simulink model "UAV_SIMULATOR_CA_2021a"  (R2024a)
settings: Solver=FixedStepAuto  StartTime=0.0  StopTime=tf_echelons  FixedStep=0.002  RelTol=1e-4
values from neighbouring files (symbols this model uses):
  Beta_OPT = [Beta, Z_max: 0.1*pi/180: betaf]    [UAV_SIMULATOR_MAIN_0.m]
  betaf = 20*pi/180 +betai    (= 0.660268528005)    [UAV_SIMULATOR_MAIN_0.m]
  betai = 17.8306*pi/180    (= 0.311202677606)    [UAV_SIMULATOR_MAIN_0.m]
  Bp_offset = 0.06    [UAV_SIMULATOR_MAIN_0.m]
  CDy = data(1)    [Aero_initial.m]    (also in FunLagragian.m; UAV_SIMULATOR_MAIN_0.m = 1; costFunction.m; nonLinearConstraints.m)
  CLOSED_LOOP_ESCs = 1    [UAV_SIMULATOR_MAIN_0.m]
  cQ = 2.1113*1e-08    (= 2.1113e-08)    [UAV_SIMULATOR_MAIN_0.m]
  cQ_Magnus = 0.5*S/2*RM^3*Cf    (= 4.804078125e-10)    [UAV_SIMULATOR_MAIN_0.m]
  cT = 2.4815e-6    (= 2.4815e-06)    [UAV_SIMULATOR_MAIN_0.m]
  cT_1_6 = 2.1030e-06    (= 2.103e-06)    [UAV_SIMULATOR_MAIN_0.m]
  D_PQR_PX4 = diag([D_ROLL D_PITCH D_YAW])    [UAV_SIMULATOR_MAIN_0.m]
  ethaf = 25*pi/180    (= 0.436332312999)    [UAV_SIMULATOR_MAIN_0.m]
  ethai = 0 *pi/180    (= 0)    [UAV_SIMULATOR_MAIN_0.m]
  F_fric = 0.5    [UAV_SIMULATOR_MAIN_0.m]
  Fa_L_int = Rmat*(FaG_int+FaG_int_d)    [UAV_SIMULATOR_MAIN_0.m]
  g = data(7)    [FunLagragian.m]    (also in UAV_SIMULATOR_MAIN_0.m = 9.81; costFunction.m; nonLinearConstraints.m; runOptimizationHelper.m = comp(7))
  I_PQR_PX4 = diag([I_ROLL I_PITCH I_YAW])    [UAV_SIMULATOR_MAIN_0.m]
  initial_attitude_condition = 1*[0 0 pi]    [UAV_SIMULATOR_MAIN_0.m]
  initial_pos_conditions = [ri*cos(betai) 0 ri*sin(betai) + Bp_offset]    [UAV_SIMULATOR_MAIN_0.m]
  Jr = 1.2991*1e-05    (= 1.2991e-05)    [UAV_SIMULATOR_MAIN_0.m]
  Jr_Magnus = JM1(2,2)    [UAV_SIMULATOR_MAIN_0.m]
  K_DI_int = [diag([k_r(1), k_etha(1), k_beta(1)]), diag([k_r(2), k_etha(2), k_beta(2)]), diag([k_r(3), k_etha(3), k_beta(3)])]    [UAV_SIMULATOR_MAIN_0.m]
  K_PQR_PX4 = 1*diag([0.8 1.35 1])    [UAV_SIMULATOR_MAIN_0.m]
  km = 1/Kv_motor_rad    (= 0.00545674090601)    [UAV_SIMULATOR_MAIN_0.m]
  L = lqr(A,B,Q_beta,R_beta)    [UAV_SIMULATOR_MAIN_0.m]
  L_mot = 1.0000e-04    (= 0.0001)    [UAV_SIMULATOR_MAIN_0.m]
  LM = 0.28*2    (= 0.56)    [UAV_SIMULATOR_MAIN_0.m]
  m = data(6)    [FunLagragian.m]    (also in UAV_SIMULATOR_MAIN_0.m = 1.746; costFunction.m; nonLinearConstraints.m; runOptimizationHelper.m = comp(6))
  m_M1 = 0.049    [UAV_SIMULATOR_MAIN_0.m]
  m_M2 = 0.049    [UAV_SIMULATOR_MAIN_0.m]
  m_w = 0.0481    [UAV_SIMULATOR_MAIN_0.m]    (also in nonLinearConstraints.m = data(9); runOptimizationHelper.m = comp(9))
  max_angle = max_angle_deg*pi/180    (= 0.610865238198)    [UAV_SIMULATOR_MAIN_0.m]
  nb_battery_cells = 4    [UAV_SIMULATOR_MAIN_0.m]
  P_ATTITUDE_PX4 = diag([10 10 2.8])    [UAV_SIMULATOR_MAIN_0.m]
  P_PQR_PX4 = diag([P_ROLL P_PITCH P_YAW])    [UAV_SIMULATOR_MAIN_0.m]
  PX4_attitude_loop_frequency = 250    [UAV_SIMULATOR_MAIN_0.m]
  PX4_rate_loop_frequency = 500    [UAV_SIMULATOR_MAIN_0.m]
  R = data(4)    [Aero_initial.m]    (also in UAV_SIMULATOR_MAIN_0.m = 0.07)
  R_bat = 0.024    [UAV_SIMULATOR_MAIN_0.m]
  rf = 1.5    [UAV_SIMULATOR_MAIN_0.m]
  rho_air = data(8)    [FunLagragian.m]    (also in UAV_SIMULATOR_MAIN_0.m = 1.293; costFunction.m; nonLinearConstraints.m; runOptimizationHelper.m = comp(8))
  ri = 0.490142    [UAV_SIMULATOR_MAIN_0.m]
  RM = data(4)    [FunLagragian.m]    (also in UAV_SIMULATOR_MAIN_0.m = 0.0275; costFunction.m; nonLinearConstraints.m; runOptimizationHelper.m = comp(4))
  S = data(3)    [Aero_initial.m]    (also in FunLagragian.m; UAV_SIMULATOR_MAIN_0.m = 0.0308; costFunction.m; nonLinearConstraints.m)
  s_M1D = [0, LM/4, 0]'    [UAV_SIMULATOR_MAIN_0.m]
  s_M2D = [0, -LM/4, 0]'    [UAV_SIMULATOR_MAIN_0.m]
  Slat = data(2)    [Aero_initial.m]    (also in FunLagragian.m; UAV_SIMULATOR_MAIN_0.m = 0.00237582944428; costFunction.m; nonLinearConstraints.m)
  state_int = [0 0 0 initial_attitude_condition 0 0 0 initial_attitude_quaternion_condition]    [UAV_SIMULATOR_MAIN_0.m]
  T0 = 1.5    [UAV_SIMULATOR_MAIN_0.m]
  t0 = 0    [UAV_SIMULATOR_MAIN_0.m]
  t1 = t0 + 15    (= 15)    [UAV_SIMULATOR_MAIN_0.m]
  t1T = t1/10    (= 1.5)    [UAV_SIMULATOR_MAIN_0.m]
  t2 = t1 + 15    (= 30)    [UAV_SIMULATOR_MAIN_0.m]    (also in plot_test.m = Simulation_Data.time)
  t2T = t2 + 9*t1/10    (= 43.5)    [UAV_SIMULATOR_MAIN_0.m]
  t3 = t2 + 15    (= 45)    [UAV_SIMULATOR_MAIN_0.m]
  tau_ur_model = 0.001    [UAV_SIMULATOR_MAIN_0.m]
  Tf = 1.5    [UAV_SIMULATOR_MAIN_0.m]
  Ti = 0    [UAV_SIMULATOR_MAIN_0.m]
  Ts = 0.02    [UAV_SIMULATOR_MAIN_0.m]
  U_sat = 3.7*nb_battery_cells    (= 14.8)    [UAV_SIMULATOR_MAIN_0.m]
  ViconTracker_noise_mean = 0.00001    (= 1e-05)    [UAV_SIMULATOR_MAIN_0.m]
  ViconTracker_noise_variance = 0.000001    (= 1e-06)    [UAV_SIMULATOR_MAIN_0.m]
  vitesse_vent = [0, 0, 0]'    [UAV_SIMULATOR_MAIN_0.m]
  vmag = 0    [UAV_SIMULATOR_MAIN_0.m]
  vx_wind = [vwind(1,1:t_winddirc_change/dt-1) vx_inter vwind(1,(t_winddirc_change+1)/dt +1:final_time/dt+1)*cos(10*pi/180)]    [UAV_SIMULATOR_MAIN_0.m]
  vy_wind = [zeros(1,t_winddirc_change/dt-1) vy_inter vwind(1,(t_winddirc_change+1)/dt +1:final_time/dt+1)*sin(10*pi/180)]    [UAV_SIMULATOR_MAIN_0.m]
  wind_turb = 1    [UAV_SIMULATOR_MAIN_0.m]
  wn_beta = 2    [UAV_SIMULATOR_MAIN_0.m]
  wn_etha = 2    [UAV_SIMULATOR_MAIN_0.m]
  wn_r = 2    [UAV_SIMULATOR_MAIN_0.m]
  X0 = 4    [UAV_SIMULATOR_MAIN_0.m]    (also in runOptimizationHelper.m = data(19))
  X1 = min(X1,8)    [Aero_initial.m]    (also in UAV_SIMULATOR_MAIN_0.m = [X1, X1(end)])
undefined symbols (not defined in the file or in its folder): DiscIntNeverNeededParam, PWM_data_map
libraries: simulink x23, slpidlib x5, eeGeneralControl x3, simulink_extras x1
(part 2 of 3)

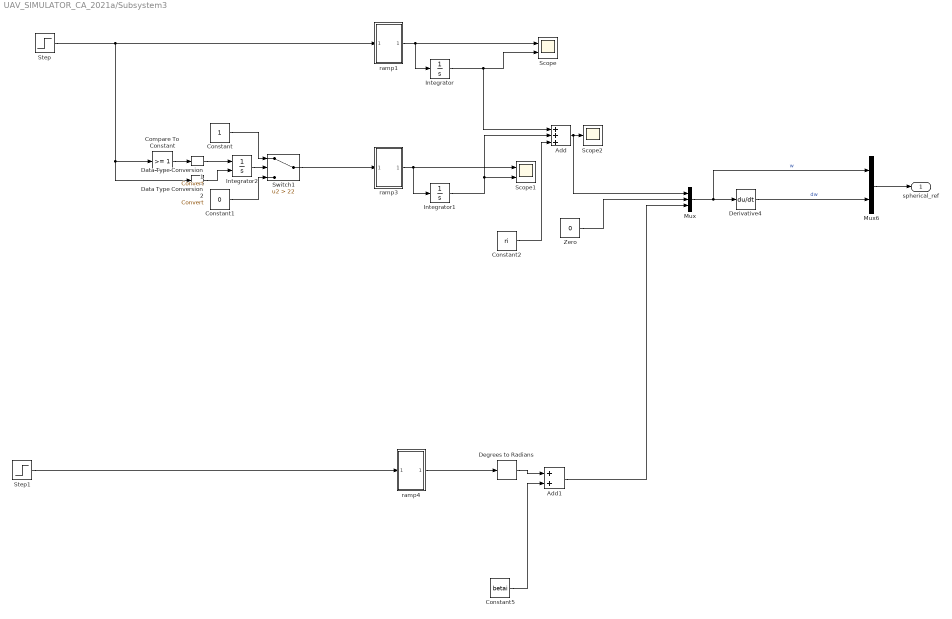
== system UAV_SIMULATOR_CA_2021a/Subsystem3 ==
  Add : Sum  Inputs=+++
  Add1 : Sum
  Compare To Constant : simulink/Logic and Bit Operations/Compare To Constant  relop=>=  const=1  OutDataTypeStr=uint8
  Constant : Constant
  Constant1 : Constant  Value=0
  Constant2 : Constant  Value=ri
  Constant5 : Constant  Value=betai
  Data Type Conversion1 : DataTypeConversion  SaturateOnIntegerOverflow=off  RndMeth=Floor
  Data Type Conversion2 : DataTypeConversion  SaturateOnIntegerOverflow=off  RndMeth=Floor
  Degrees to Radians : simulink_extras/Transformations/Degrees to Radians
  Derivative4 : Derivative
  Integrator : Integrator
  Integrator1 : Integrator
  Integrator2 : Integrator  ExternalReset=falling
  Mux : Mux  Inputs=3
  Mux6 : Mux  Inputs=2
  Scope : Scope  NumInputPorts=2
  Scope1 : Scope  NumInputPorts=2
  Scope2 : Scope
  Step : Step  Time=0  SampleTime=0
  Step1 : Step  Time=0  SampleTime=0
  Switch1 : Switch  Criteria=u2 > Threshold  Threshold=22  SaturateOnIntegerOverflow=off  InputSameDT=off
  Zero : Constant  Value=0  OutDataTypeStr=Inherit: Inherit via back propagation
  ramp1 : Subsystem  mask{tf1=4, tf2=8, tf3=4, g1=(1/12)/4, g2=(1/12)/4}
      mask prompts: tf1 "temps fin rampe montante"; tf2 "temps fin constante"; tf3 "temps fin rampe descendente"; g1 "gain rampe 1"; g2 "gain rampe 2"
  ramp3 : Subsystem  mask{tf1=4, tf2=8, tf3=4, g1=-(1/12)/4, g2=-(1/12)/4}
      mask prompts: tf1 "temps fin rampe montante"; tf2 "temps fin constante"; tf3 "temps fin rampe descendente"; g1 "gain rampe 1"; g2 "gain rampe 2"
  ramp4 : Subsystem  mask{tf1=10, tf2=26, tf3=10, g1=15/10, g2=15/10}
      mask prompts: tf1 "temps fin rampe montante"; tf2 "temps fin constante"; tf3 "temps fin rampe descendente"; g1 "gain rampe 1"; g2 "gain rampe 2"
  spherical_ref : Outport
  wires:
  Degrees to Radians/1 -> Add1/1
  ramp3/1(Out1) -> Scope1/1, Integrator1/1
  ramp4/1(Out1) -> Degrees to Radians/1
  Constant1/1 -> Switch1/3
  Constant/1 -> Switch1/1
  ramp1/1(Out1) -> Scope/1, Integrator/1
  Add/1 -> Mux/1, Scope2/1
  Compare To Constant/1 -> Data Type Conversion1/1
  Switch1/1 -> ramp3/1(In1)
  Integrator2/1 -> Switch1/2
  Data Type Conversion2/1 -> Integrator2/2
  Data Type Conversion1/1 -> Integrator2/1
  Integrator1/1 -> Scope1/2, Add/2
  Step/1 -> ramp1/1(In1), Compare To Constant/1, Data Type Conversion2/1
  Constant2/1 -> Add/3
  Integrator/1 -> Scope/2, Add/1
  Constant5/1 -> Add1/2
  Add1/1 -> Mux/3
  Zero/1 -> Mux/2
  Mux6/1 -> spherical_ref/1
  Mux/1 -> Derivative4/1, Mux6/1  "w"
  Derivative4/1 -> Mux6/2  "dw"
  Step1/1 -> ramp4/1(In1)

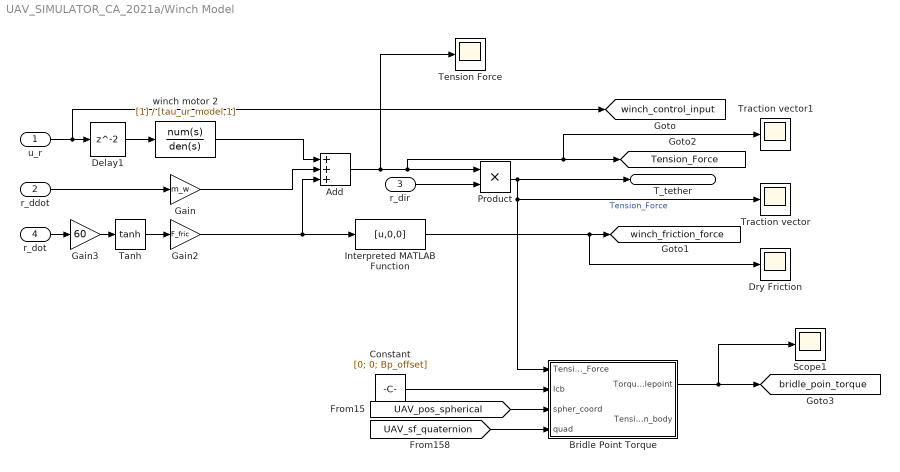
== system UAV_SIMULATOR_CA_2021a/Winch Model ==
  u_r : Inport
  r_ddot : Inport  Port=2
  r_dir : Inport  Port=3
  r_dot : Inport  Port=4
  Add : Sum  Inputs=+++
  Bridle Point Torque : MATLAB Function  TreatAsAtomicUnit=on
  Constant : Constant  Value=[0; 0; Bp_offset]
  Delay1 : Delay  SampleTime=Ts
  Dry Friction : Scope
  Gain : Gain  Gain=m_w
  Gain2 : Gain  Gain=F_fric
  Gain3 : Gain  Gain=60
  Interpreted MATLAB Function : MATLABFcn  MATLABFcn=[u,0,0]
  Product : Product
  Scope1 : Scope
  Tanh : Trigonometry  Operator=tanh
  Tension Force : Scope
  Traction vector : Scope
  Traction vector1 : Scope
  winch motor 2 : TransferFcn  Denominator=[tau_ur_model,1]
  T_tether : Outport
  tag scope: Tension_Force=global, bridle_poin_torque=global, winch_control_input=global, winch_friction_force=global
  wires:
  Gain/1 -> Add/2
  Product/1 -> T_tether/1, Traction vector/1, Bridle Point Torque/1(Tension_Force)  "Tension_Force"
  Add/1 -> Tension Force/1, Traction vector1/1, [Tension_Force], Product/1
  r_dir/1 -> Product/2
  r_dot/1 -> Gain3/1
  Interpreted MATLAB Function/1 -> Dry Friction/1, [winch_friction_force]
  Tanh/1 -> Gain2/1
  Gain3/1 -> Tanh/1
  r_ddot/1 -> Gain/1
  u_r/1 -> [winch_control_input], Delay1/1
  Gain2/1 -> Interpreted MATLAB Function/1, Add/3
  Delay1/1 -> winch motor 2/1
  winch motor 2/1 -> Add/1
  Constant/1 -> Bridle Point Torque/2(lcb)
  [UAV_pos_spherical] -> Bridle Point Torque/3(spher_coord)
  [UAV_sf_quaternion] -> Bridle Point Torque/4(quad)
  Bridle Point Torque/1(Torque_bridlepoint) -> Scope1/1, [bridle_poin_torque]

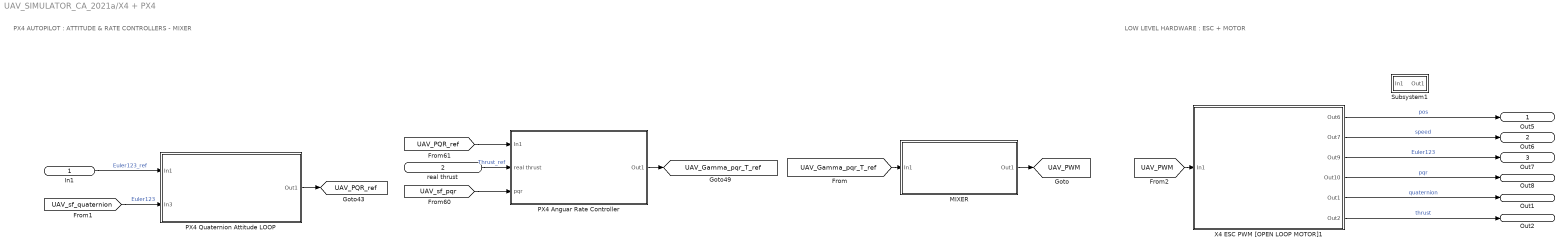
== system UAV_SIMULATOR_CA_2021a/X4 + PX4  ==
  note: LOW LEVEL HARDWARE : ESC + MOTOR
  note: PX4 AUTOPILOT : ATTITUDE & RATE CONTROLLERS - MIXER
  In1 : Inport
  real thrust : Inport  Port=2
  MIXER : Subsystem
  PX4 Anguar Rate Controller : Subsystem
  PX4 Quaternion Attitude LOOP : Subsystem
  Subsystem1 : Subsystem
  X4 ESC PWM [OPEN LOOP MOTOR]1 : Subsystem
  Out5 : Outport
  Out6 : Outport  Port=2
  Out7 : Outport  Port=3
  Out8 : Outport  Port=4
  Out1 : Outport  Port=5
  Out2 : Outport  Port=6
  tag scope: UAV_Gamma_pqr_T_ref=global, UAV_PQR_ref=global, UAV_PWM=global
  wires:
  [UAV_sf_quaternion] -> PX4 Quaternion Attitude LOOP/2(In3)  "Euler123"
  PX4 Quaternion Attitude LOOP/1(Out1) -> [UAV_PQR_ref]
  [UAV_Gamma_pqr_T_ref] -> MIXER/1(In1)
  [UAV_sf_pqr] -> PX4 Anguar Rate Controller/3(pqr)
  MIXER/1(Out1) -> [UAV_PWM]
  real thrust/1 -> PX4 Anguar Rate Controller/2(real thrust)  "Thrust_ref"
  In1/1 -> PX4 Quaternion Attitude LOOP/1(In1)  "Euler123_ref"
  [UAV_PQR_ref] -> PX4 Anguar Rate Controller/1(In1)
  PX4 Anguar Rate Controller/1(Out1) -> [UAV_Gamma_pqr_T_ref]
  X4 ESC PWM [OPEN LOOP MOTOR]1/3(Out9) -> Out7/1  "Euler123"
  X4 ESC PWM [OPEN LOOP MOTOR]1/2(Out7) -> Out6/1  "speed"
  [UAV_PWM] -> X4 ESC PWM [OPEN LOOP MOTOR]1/1(In1)
  X4 ESC PWM [OPEN LOOP MOTOR]1/4(Out10) -> Out8/1  "pqr"
  X4 ESC PWM [OPEN LOOP MOTOR]1/5(Out1) -> Out1/1  "quaternion"
  X4 ESC PWM [OPEN LOOP MOTOR]1/6(Out2) -> Out2/1  "thrust"
  X4 ESC PWM [OPEN LOOP MOTOR]1/1(Out6) -> Out5/1  "pos"

== system UAV_SIMULATOR_CA_2021a/r_ref ==
  Add : Sum  Inputs=+++
  Add1 : Sum  Inputs=+++
  Add3 : Sum
  Add4 : Sum  Inputs=+++
  Ramp : simulink/Sources/Ramp  slope=(Tf-Ti)/(t1T-t0)  start=t0  InitialOutput=Ti
  Ramp2 : simulink/Sources/Ramp  slope=-(Tf-Ti)/(t1T-t0)  start=t1T  InitialOutput=-Tf
  Ramp3 : simulink/Sources/Ramp  slope=(Ti-Tf)/(t3-t2T)  start=t2T  InitialOutput=Tf
  Ramp5 : simulink/Sources/Ramp  slope=-(Ti-Tf)/(t3-t2T)  start=t3  InitialOutput=-Ti  VectorParams1D=off
  Step : Step  Time=t2T  Before=Tf  After=0  SampleTime=0
  Step2 : Step  Time=t1T  Before=-Tf  After=0  SampleTime=0
  Step4 : Step  Time=t1T  Before=Tf  After=0  SampleTime=0
  Step6 : Step  Time=t2T  Before=Ti-Tf  After=Ti  SampleTime=0
  T_ref : Outport
  wires:
  Add3/1 -> Add4/2
  Ramp/1 -> Add/1
  Step6/1 -> Add1/3
  Ramp2/1 -> Add/2
  Ramp3/1 -> Add1/1
  Add1/1 -> Add4/3
  Add4/1 -> T_ref/1
  Step/1 -> Add3/1
  Ramp5/1 -> Add1/2
  Step2/1 -> Add3/2
  Step4/1 -> Add/3
  Add/1 -> Add4/1

== system UAV_SIMULATOR_CA_2021a/ramp4 ==
  In1 : Inport
  Add : Sum
  Compare To Constant : simulink/Logic and Bit Operations/Compare To Constant  relop=>=  const=1  OutDataTypeStr=uint8
  Constant : Constant  Value=-1
  Constant1 : Constant  Value=0
  Data Type Conversion1 : DataTypeConversion  SaturateOnIntegerOverflow=off  RndMeth=Floor
  Data Type Conversion2 : DataTypeConversion  SaturateOnIntegerOverflow=off  RndMeth=Floor
  Gain : Gain  Gain=g1
  Gain2 : Gain  Gain=g2
  Integrator : Integrator  ExternalReset=falling
  Integrator1 : Integrator  ExternalReset=falling
  Switch : Switch  Criteria=u2 > Threshold  Threshold=tf2+tf1  SaturateOnIntegerOverflow=off  InputSameDT=off
  Switch1 : Switch  Criteria=u2 > Threshold  Threshold=tf1  SaturateOnIntegerOverflow=off  InputSameDT=off
  Switch2 : Switch  Criteria=u2 > Threshold  Threshold=tf3+tf2+tf1  SaturateOnIntegerOverflow=off  InputSameDT=off
  Out1 : Outport
  wires:
  Compare To Constant/1 -> Data Type Conversion1/1
  Integrator/1 -> Switch1/2, Switch2/2, Switch/2
  In1/1 -> Data Type Conversion2/1, Compare To Constant/1
  Data Type Conversion1/1 -> Integrator/1, Switch1/3
  Data Type Conversion2/1 -> Integrator1/2, Integrator/2
  Constant/1 -> Switch/1
  Switch2/1 -> Gain2/1
  Constant1/1 -> Switch/3, Switch2/1, Switch1/1
  Switch1/1 -> Gain/1
  Integrator1/1 -> Out1/1
  Gain2/1 -> Add/2
  Gain/1 -> Add/1
  Add/1 -> Integrator1/1
  Switch/1 -> Switch2/3

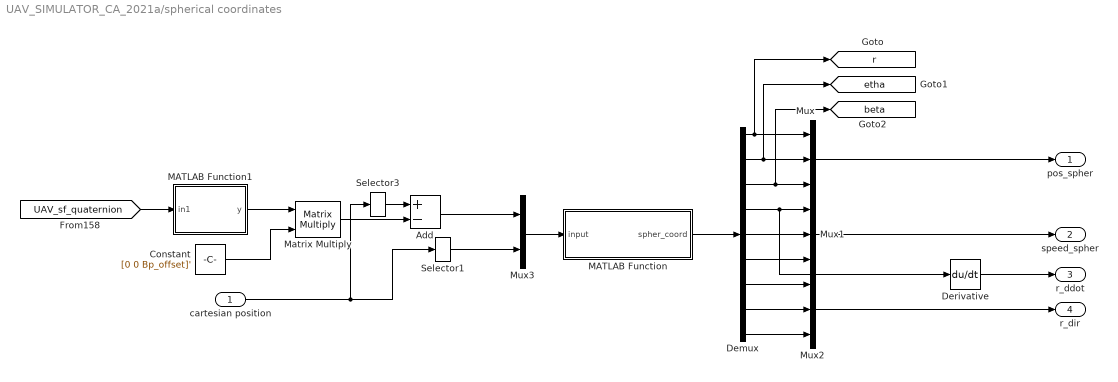
== system UAV_SIMULATOR_CA_2021a/spherical coordinates ==
  "cartesian position " : Inport
  Add : Sum  Inputs=+-
  Constant : Constant  Value=[0 0 Bp_offset]'
  Demux : Demux  Outputs=9
  Derivative : Derivative
  MATLAB Function : MATLAB Function  TreatAsAtomicUnit=on
  MATLAB Function1 : MATLAB Function  TreatAsAtomicUnit=on
  Matrix Multiply : Product  Multiplication=Matrix(*)
  Mux : Mux  Inputs=3
  Mux1 : Mux  Inputs=3
  Mux2 : Mux  Inputs=3
  Mux3 : Mux  Inputs=2
  Selector1 : Selector  InputPortWidth=6  IndexOptions=Index vector (dialog)  Indices=[4:6]  OutputSizes=1
  Selector3 : Selector  InputPortWidth=6  IndexOptions=Index vector (dialog)  Indices=[1:3]  OutputSizes=1
  pos_spher : Outport
  speed_spher : Outport  Port=2
  r_ddot : Outport  Port=3
  r_dir : Outport  Port=4
  tag scope: beta=global, etha=global, r=global
  wires:
  MATLAB Function/1(spher_coord) -> Demux/1
  Demux/1 -> [r], Mux/1
  Demux/2 -> [etha], Mux/2
  Demux/3 -> [beta], Mux/3
  Demux/5 -> Mux1/2
  Demux/6 -> Mux1/3
  Demux/4 -> Derivative/1, Mux1/1
  Mux/1 -> pos_spher/1
  Mux1/1 -> speed_spher/1
  Derivative/1 -> r_ddot/1
  Demux/7 -> Mux2/1
  Demux/8 -> Mux2/2
  Demux/9 -> Mux2/3
  Mux2/1 -> r_dir/1
  Selector3/1 -> Add/1
  "cartesian position "/1 -> Selector1/1, Selector3/1
  Constant/1 -> Matrix Multiply/2
  Matrix Multiply/1 -> Add/2
  MATLAB Function1/1(y) -> Matrix Multiply/1
  [UAV_sf_quaternion] -> MATLAB Function1/1(in1)
  Selector1/1 -> Mux3/2
  Add/1 -> Mux3/1
  Mux3/1 -> MATLAB Function/1(input)

== system UAV_SIMULATOR_CA_2021a/Aerodynamic Forces/Magnus_Actuator ==
  In1 : Inport
  PID Controller1 : slpidlib/PID Controller  Controller=PID  Form=Parallel  TimeDomain=Continuous-time  UseExternalTs=off  SampleTime=-1  IntegratorMethod=Forward Euler  FilterMethod=Forward Euler  ControllerParametersSource=internal  P=0.01  I=0.4  UseKiTs=off  D=0  UseExternalDerivativeSource=off  N=100  UseFilter=on  TunerSelectOption=Transfer Function Based (PID Tuner App)  InitialConditionSource=internal  InitialConditionForIntegrator=0  InitialConditionForFilter=0  DifferentiatorICPrevScaledInput=0  ExternalReset=none  TrackingMode=off  Kt=1  LimitOutput=off  SatLimitsSource=internal  UpperSaturationLimit=inf  LowerSaturationLimit=-inf  LinearizeAsGain=on  AntiWindupMode=none  Kb=1  LimitIntegrator=off  UpperIntegratorSaturationLimit=inf  LowerIntegratorSaturationLimit=-inf  POutMin=[]  POutMax=[]  IOutMin=[]  IOutMax=[]  DOutMin=[]  DOutMax=[]  NOutMin=[]  NOutMax=[]  SumOutMin=[]  SumOutMax=[]  SaturationOutMin=[]  SaturationOutMax=[]  PParamMin=[]  PParamMax=[]  IParamMin=[]  IParamMax=[]  DParamMin=[]  DParamMax=[]  NParamMin=[]  NParamMax=[]  KbParamMin=[]  KbParamMax=[]  KtParamMin=[]  KtParamMax=[]  KbOutMin=[]  KbOutMax=[]  KtOutMin=[]  KtOutMax=[]  IntegratorOutMin=[]  IntegratorOutMax=[]  FilterOutMin=[]  FilterOutMax=[]  SumI1OutMin=[]  SumI1OutMax=[]  SumI2OutMin=[]  SumI2OutMax=[]  SumI3OutMin=[]  SumI3OutMax=[]  SumI4OutMin=[]  SumI4OutMax=[]  SumDOutMin=[]  SumDOutMax=[]  DifferentiatorOutMin=[]  DifferentiatorOutMax=[]  FilterDiffOutCoefMin=[]  FilterDiffOutCoefMax=[]  ReciprocalOutMin=[]  ReciprocalOutMax=[]  SumDenOutMin=[]  SumDenOutMax=[]  SumNumOutMin=[]  SumNumOutMax=[]  DivideOutMin=[]  DivideOutMax=[]  UdiffTsProdOutMin=[]  UdiffTsProdOutMax=[]  NTsProdOutMin=[]  NTsProdOutMax=[]  UintegralTsProdOutMin=[]  UintegralTsProdOutMax=[]  UngainTsProdOutMin=[]  UngainTsProdOutMax=[]  ClampingZeroOutDataTypeStr=Inherit: Inherit via back propagation  ClampingZeroOutMin=[]  ClampingZeroOutMax=[]  FilterDenConstantOutDataTypeStr=Inherit: Inherit via back propagation  FilterDenConstantOutMin=[]  FilterDenConstantOutMax=[]  PCopyOutDataTypeStr=Inherit: Inherit via back propagation  PCopyOutMin=[]  PCopyOutMax=[]  NCopyOutDataTypeStr=Inherit: Inherit via back propagation  NCopyOutMin=[]  NCopyOutMax=[]  IntegratorContinuousStateAttributes=''  IntegratorStateMustResolveToSignalObject=off  IntegratorRTWStateStorageClass=Auto  FilterContinuousStateAttributes=''  FilterStateMustResolveToSignalObject=off  FilterRTWStateStorageClass=Auto  ParallelPVariant=InternalParameters  IdealPVariant=Disabled  IVariant=InternalParameters  DVariant=InternalParameters  IntegratorVariant=Continuous  SatVariant=Disabled  AWVariant=Passthrough  PCopyVariant=Disabled  TRVariant=Disabled  FdbkBlocksVariant=Forward  IdealPFdbkVariant=Disabled  SatFdbkVariant=Disabled  DerivativeFilterVariant=ContFilter  NVariant=InternalParameters  NCopyVariant=Disabled  FilterICVariant=InternalICsFilter  IntegratorICVariant=InternalICs  ExternalResetVariant=Disabled  TRSumVariant=Passthrough  SumFdbkVariant=Disabled  SumVariant=Sum_PID  TsampFilterVariant=InternalTs  TsampNgainVariant=Passthrough  TsampIntegralVariant=Disabled_SignalSpec  ExternalSaturationOutDataTypeStr=Inherit: Same as second input  DerivativeSourceVariant=ErrorSignal
  Scope : Scope
  Subsystem : Subsystem
  Sum7 : Sum  Inputs=|+-
  motor_speed : Outport
  wires:
  Sum7/1 -> PID Controller1/1
  In1/1 -> Scope/1, Sum7/1  "rotation_speed"
  PID Controller1/1 -> Subsystem/1(In1)
  Subsystem/1(Out1) -> motor_speed/1, Sum7/2  "motor_speed"

== system UAV_SIMULATOR_CA_2021a/Subsystem1/beta_ref ==
  Add10 : Sum
  Add11 : Sum  Inputs=+++
  Add8 : Sum  Inputs=+++
  Add9 : Sum  Inputs=+++
  Ramp10 : simulink/Sources/Ramp  slope=(betai-betaf)/(t3-t2)  start=t2  InitialOutput=betaf
  Ramp11 : simulink/Sources/Ramp  slope=-(betai-betaf)/(t3-t2)  start=t3  InitialOutput=-betai  VectorParams1D=off
  Ramp8 : simulink/Sources/Ramp  slope=(betaf-betai)/(t1-t0)  start=t0  InitialOutput=betai
  Ramp9 : simulink/Sources/Ramp  slope=-(betaf-betai)/(t1-t0)  start=t1  InitialOutput=-betaf
  Step10 : Step  Time=t1  Before=betaf  After=0  SampleTime=0
  Step11 : Step  Time=t2  Before=betai-betaf  After=betai  SampleTime=0
  Step8 : Step  Time=t2  Before=betaf  After=0  SampleTime=0
  Step9 : Step  Time=t1  Before=-betaf  After=0  SampleTime=0
  beta-ref : Outport
  wires:
  Ramp10/1 -> Add9/1
  Ramp11/1 -> Add9/2
  Ramp8/1 -> Add8/1
  Step11/1 -> Add9/3
  Add9/1 -> Add11/3
  Add11/1 -> beta-ref/1
  Step10/1 -> Add8/3
  Step8/1 -> Add10/1
  Add10/1 -> Add11/2
  Step9/1 -> Add10/2
  Add8/1 -> Add11/1
  Ramp9/1 -> Add8/2

== system UAV_SIMULATOR_CA_2021a/Subsystem1/etha_ref1 ==
  Add10 : Sum
  Add11 : Sum  Inputs=+++
  Add8 : Sum  Inputs=+++
  Add9 : Sum  Inputs=+++
  Ramp10 : simulink/Sources/Ramp  slope=(ethai-ethaf)/(t3-t2)  start=t2  InitialOutput=ethaf
  Ramp11 : simulink/Sources/Ramp  slope=-(ethai-ethaf)/(t3-t2)  start=t3  InitialOutput=-ethai  VectorParams1D=off
  Ramp8 : simulink/Sources/Ramp  slope=(ethaf-ethai)/(t1-t0)  start=t0  InitialOutput=ethai
  Ramp9 : simulink/Sources/Ramp  slope=-(ethaf-ethai)/(t1-t0)  start=t1  InitialOutput=-ethaf
  Step10 : Step  Time=t1  Before=ethaf  After=0  SampleTime=0
  Step11 : Step  Time=t2  Before=ethai-ethaf  After=ethai  SampleTime=0
  Step8 : Step  Time=t2  Before=ethaf  After=0  SampleTime=0
  Step9 : Step  Time=t1  Before=-ethaf  After=0  SampleTime=0
  beta-ref : Outport
  wires:
  Ramp10/1 -> Add9/1
  Ramp11/1 -> Add9/2
  Ramp8/1 -> Add8/1
  Step11/1 -> Add9/3
  Add9/1 -> Add11/3
  Add11/1 -> beta-ref/1  "etha_ref"
  Step10/1 -> Add8/3
  Step8/1 -> Add10/1
  Add10/1 -> Add11/2
  Step9/1 -> Add10/2
  Add8/1 -> Add11/1
  Ramp9/1 -> Add8/2

== system UAV_SIMULATOR_CA_2021a/Subsystem1/r_ref ==
  Add : Sum  Inputs=+++
  Add1 : Sum  Inputs=+++
  Add3 : Sum
  Add4 : Sum  Inputs=+++
  Ramp : simulink/Sources/Ramp  slope=(rf-ri)/(t1-t0)  start=t0  InitialOutput=ri
  Ramp2 : simulink/Sources/Ramp  slope=-(rf-ri)/(t1-t0)  start=t1  InitialOutput=-rf
  Ramp3 : simulink/Sources/Ramp  slope=(ri-rf)/(t3-t2)  start=t2  InitialOutput=rf
  Ramp5 : simulink/Sources/Ramp  slope=-(ri-rf)/(t3-t2)  start=t3  InitialOutput=-ri  VectorParams1D=off
  Step : Step  Time=t2  Before=rf  After=0  SampleTime=0
  Step2 : Step  Time=t1  Before=-rf  After=0  SampleTime=0
  Step4 : Step  Time=t1  Before=rf  After=0  SampleTime=0
  Step6 : Step  Time=t2  Before=ri-rf  After=ri  SampleTime=0
  r_ref : Outport
  wires:
  Add3/1 -> Add4/2
  Ramp/1 -> Add/1
  Step6/1 -> Add1/3
  Ramp2/1 -> Add/2
  Ramp3/1 -> Add1/1
  Add1/1 -> Add4/3
  Add4/1 -> r_ref/1
  Step/1 -> Add3/1
  Ramp5/1 -> Add1/2
  Step2/1 -> Add3/2
  Step4/1 -> Add/3
  Add/1 -> Add4/1

== system UAV_SIMULATOR_CA_2021a/Subsystem3/ramp1 ==
  In1 : Inport
  Add : Sum
  Compare To Constant : simulink/Logic and Bit Operations/Compare To Constant  relop=>=  const=1  OutDataTypeStr=uint8
  Constant : Constant  Value=-1
  Constant1 : Constant  Value=0
  Data Type Conversion1 : DataTypeConversion  SaturateOnIntegerOverflow=off  RndMeth=Floor
  Data Type Conversion2 : DataTypeConversion  SaturateOnIntegerOverflow=off  RndMeth=Floor
  Gain : Gain  Gain=g1
  Gain2 : Gain  Gain=g2
  Integrator : Integrator  ExternalReset=falling
  Integrator1 : Integrator  ExternalReset=falling
  Switch : Switch  Criteria=u2 > Threshold  Threshold=tf2+tf1  SaturateOnIntegerOverflow=off  InputSameDT=off
  Switch1 : Switch  Criteria=u2 > Threshold  Threshold=tf1  SaturateOnIntegerOverflow=off  InputSameDT=off
  Switch2 : Switch  Criteria=u2 > Threshold  Threshold=tf3+tf2+tf1  SaturateOnIntegerOverflow=off  InputSameDT=off
  Out1 : Outport
  wires:
  Compare To Constant/1 -> Data Type Conversion1/1
  Integrator/1 -> Switch1/2, Switch2/2, Switch/2
  In1/1 -> Data Type Conversion2/1, Compare To Constant/1
  Data Type Conversion1/1 -> Integrator/1, Switch1/3
  Data Type Conversion2/1 -> Integrator1/2, Integrator/2
  Constant/1 -> Switch/1
  Switch2/1 -> Gain2/1
  Constant1/1 -> Switch/3, Switch2/1, Switch1/1
  Switch1/1 -> Gain/1
  Integrator1/1 -> Out1/1
  Gain2/1 -> Add/2
  Gain/1 -> Add/1
  Add/1 -> Integrator1/1
  Switch/1 -> Switch2/3

== system UAV_SIMULATOR_CA_2021a/Subsystem3/ramp3 ==
  In1 : Inport
  Add : Sum
  Compare To Constant : simulink/Logic and Bit Operations/Compare To Constant  relop=>=  const=1  OutDataTypeStr=uint8
  Constant : Constant  Value=-1
  Constant1 : Constant  Value=0
  Data Type Conversion1 : DataTypeConversion  SaturateOnIntegerOverflow=off  RndMeth=Floor
  Data Type Conversion2 : DataTypeConversion  SaturateOnIntegerOverflow=off  RndMeth=Floor
  Gain : Gain  Gain=g1
  Gain2 : Gain  Gain=g2
  Integrator : Integrator  ExternalReset=falling
  Integrator1 : Integrator  ExternalReset=falling
  Switch : Switch  Criteria=u2 > Threshold  Threshold=tf2+tf1  SaturateOnIntegerOverflow=off  InputSameDT=off
  Switch1 : Switch  Criteria=u2 > Threshold  Threshold=tf1  SaturateOnIntegerOverflow=off  InputSameDT=off
  Switch2 : Switch  Criteria=u2 > Threshold  Threshold=tf3+tf2+tf1  SaturateOnIntegerOverflow=off  InputSameDT=off
  Out1 : Outport
  wires:
  Switch/1 -> Switch2/3
  Add/1 -> Integrator1/1
  Gain/1 -> Add/1
  Gain2/1 -> Add/2
  Integrator1/1 -> Out1/1
  Switch1/1 -> Gain/1
  Constant1/1 -> Switch1/1, Switch2/1, Switch/3
  Switch2/1 -> Gain2/1
  Constant/1 -> Switch/1
  Data Type Conversion2/1 -> Integrator/2, Integrator1/2
  Data Type Conversion1/1 -> Switch1/3, Integrator/1
  In1/1 -> Compare To Constant/1, Data Type Conversion2/1
  Integrator/1 -> Switch/2, Switch2/2, Switch1/2
  Compare To Constant/1 -> Data Type Conversion1/1

== system UAV_SIMULATOR_CA_2021a/Subsystem3/ramp4 ==
  In1 : Inport
  Add : Sum
  Compare To Constant : simulink/Logic and Bit Operations/Compare To Constant  relop=>=  const=1  OutDataTypeStr=uint8
  Constant : Constant  Value=-1
  Constant1 : Constant  Value=0
  Data Type Conversion1 : DataTypeConversion  SaturateOnIntegerOverflow=off  RndMeth=Floor
  Data Type Conversion2 : DataTypeConversion  SaturateOnIntegerOverflow=off  RndMeth=Floor
  Gain : Gain  Gain=g1
  Gain2 : Gain  Gain=g2
  Integrator : Integrator  ExternalReset=falling
  Integrator1 : Integrator  ExternalReset=falling
  Switch : Switch  Criteria=u2 > Threshold  Threshold=tf2+tf1  SaturateOnIntegerOverflow=off  InputSameDT=off
  Switch1 : Switch  Criteria=u2 > Threshold  Threshold=tf1  SaturateOnIntegerOverflow=off  InputSameDT=off
  Switch2 : Switch  Criteria=u2 > Threshold  Threshold=tf3+tf2+tf1  SaturateOnIntegerOverflow=off  InputSameDT=off
  Out1 : Outport
  wires:
  Compare To Constant/1 -> Data Type Conversion1/1
  Integrator/1 -> Switch1/2, Switch2/2, Switch/2
  In1/1 -> Data Type Conversion2/1, Compare To Constant/1
  Data Type Conversion1/1 -> Integrator/1, Switch1/3
  Data Type Conversion2/1 -> Integrator1/2, Integrator/2
  Constant/1 -> Switch/1
  Switch2/1 -> Gain2/1
  Constant1/1 -> Switch/3, Switch2/1, Switch1/1
  Switch1/1 -> Gain/1
  Integrator1/1 -> Out1/1
  Gain2/1 -> Add/2
  Gain/1 -> Add/1
  Add/1 -> Integrator1/1
  Switch/1 -> Switch2/3

== system UAV_SIMULATOR_CA_2021a/X4 + PX4 /MIXER ==
  In1 : Inport
  Manual Switch7 : ManualSwitch  CurrentSetting=0
  PX4_controller_mixer : MATLABFcn  MATLABFcn=PX4_controller_mixer  OutputDimensions=4
  Zero-Order Hold : ZeroOrderHold  SampleTime=1/PX4_rate_loop_frequency
  controller_mixer 2 : MATLABFcn  MATLABFcn=controller_mixer  OutputDimensions=4
  Out1 : Outport
  wires:
  Manual Switch7/1 -> Out1/1  "PWMi"
  controller_mixer 2/1 -> Manual Switch7/1  "PWM"
  Zero-Order Hold/1 -> PX4_controller_mixer/1, controller_mixer 2/1  "[Gamma_pqr T]"
  PX4_controller_mixer/1 -> Manual Switch7/2  "PWM"
  In1/1 -> Zero-Order Hold/1  "[Gamma_pqr T]"

== system UAV_SIMULATOR_CA_2021a/X4 + PX4 /PX4 Anguar Rate Controller ==
  In1 : Inport
  real thrust : Inport  Port=2
  pqr : Inport  Port=3
  Discrete Derivative : simulink/Discrete/Discrete Derivative  gainval=1.0  ICPrevScaledInput=0.0  OutMin=[]  OutMax=[]  OutDataType=fixdt(1, 16)  OutScaling=2^-10  DoSatur=off
  Discrete-Time Integrator : DiscreteIntegrator  SampleTime=1/PX4_rate_loop_frequency  ICPrevOutput=DiscIntNeverNeededParam  ICPrevScaledInput=DiscIntNeverNeededParam
  Gain12 : Gain  Gain=-D_PQR_PX4  Multiplication=Matrix(K*u) (u vector)
  Gain13 : Gain  Gain=K_PQR_PX4  Multiplication=Matrix(K*u) (u vector)
  Gain14 : Gain  Gain=I_PQR_PX4  Multiplication=Matrix(K*u) (u vector)
  Gain2 : Gain  Gain=P_PQR_PX4  Multiplication=Matrix(K*u) (u vector)
  Gain7 : Gain  Gain=K_PQR_PX4  Multiplication=Matrix(K*u) (u vector)
  Mux11 : Mux  Inputs=2
  Sum1 : Sum  Inputs=+++
  Sum11 : Sum  Inputs=|+-
  Zero-Order Hold1 : ZeroOrderHold  SampleTime=1/PX4_rate_loop_frequency
  Zero-Order Hold2 : ZeroOrderHold  SampleTime=1/PX4_rate_loop_frequency
  Zero-Order Hold3 : ZeroOrderHold  SampleTime=1/PX4_rate_loop_frequency
  Out1 : Outport  VectorParamsAs1DForOutWhenUnconnected=off
  wires:
  Gain13/1 -> Discrete-Time Integrator/1, Gain2/1
  Gain2/1 -> Sum1/1
  Gain12/1 -> Sum1/3  "u = [Gamma_p Gamma_q Gamma_r]'"
  Sum11/1 -> Gain13/1
  Discrete Derivative/1 -> Gain12/1
  Sum1/1 -> Mux11/1  "u = [Gamma_p Gamma_q Gamma_r]'"
  pqr/1 -> Zero-Order Hold2/1  "pqr"
  Discrete-Time Integrator/1 -> Gain14/1
  Gain14/1 -> Sum1/2
  Gain7/1 -> Discrete Derivative/1  "u = [Gamma_p Gamma_q Gamma_r]'"
  In1/1 -> Zero-Order Hold1/1  "pqr_ref"
  real thrust/1 -> Zero-Order Hold3/1  "thrust"
  Mux11/1 -> Out1/1  "[Gamma_pqr T]"
  Zero-Order Hold1/1 -> Sum11/1
  Zero-Order Hold2/1 -> Gain7/1, Sum11/2
  Zero-Order Hold3/1 -> Mux11/2

== system UAV_SIMULATOR_CA_2021a/X4 + PX4 /PX4 Quaternion Attitude LOOP ==
  In1 : Inport
  In3 : Inport  Port=2
  Demux : Demux
  Gain : Gain  Gain=2*P_ATTITUDE_PX4  Multiplication=Matrix(K*u) (u vector)
  Interpreted MATLAB Function : MATLABFcn  MATLABFcn=euler2quaternion  OutputDimensions=4
  Mux : Mux  Inputs=3
  Mux1 : Mux  Inputs=2
  Product : Product
  Sign : Signum
  Zero-Order Hold1 : ZeroOrderHold  SampleTime=1/PX4_attitude_loop_frequency
  Zero-Order Hold2 : ZeroOrderHold  SampleTime=1/PX4_attitude_loop_frequency
  quaternion_error_from_q_qref : MATLABFcn  MATLABFcn=quaternion_error_from_q_qref  OutputDimensions=4
  Out1 : Outport  VectorParamsAs1DForOutWhenUnconnected=off
  wires:
  In1/1 -> Zero-Order Hold2/1  "Euler123_ref"
  Interpreted MATLAB Function/1 -> Mux1/2  "quaternion_ref"
  Sign/1 -> Product/1
  Demux/1 -> Sign/1
  Demux/2 -> Mux/1
  Demux/3 -> Mux/2
  Demux/4 -> Mux/3
  quaternion_error_from_q_qref/1 -> Demux/1  "eps"
  Mux/1 -> Product/2
  Product/1 -> Gain/1
  In3/1 -> Zero-Order Hold1/1  "quaternion"
  Mux1/1 -> quaternion_error_from_q_qref/1
  Zero-Order Hold1/1 -> Mux1/1  "PQR_ref"
  Zero-Order Hold2/1 -> Interpreted MATLAB Function/1  "PQR_ref"
  Gain/1 -> Out1/1  "PQR_ref"

== system UAV_SIMULATOR_CA_2021a/X4 + PX4 /Subsystem1 ==
  In1 : Inport
  Add : Sum
  Bias1 : Bias  Bias=0.0  SaturateOnIntegerOverflow=off
  Random Number : RandomNumber  Mean=ViconTracker_noise_mean  Variance=ViconTracker_noise_variance  SampleTime=Ts
  Scope : Scope  NumInputPorts=2
  Out1 : Outport
  wires:
  Bias1/1 -> Add/1
  Add/1 -> Scope/2, Out1/1  "vicon_pose"
  In1/1 -> Bias1/1, Scope/1  "pos"
  Random Number/1 -> Add/2

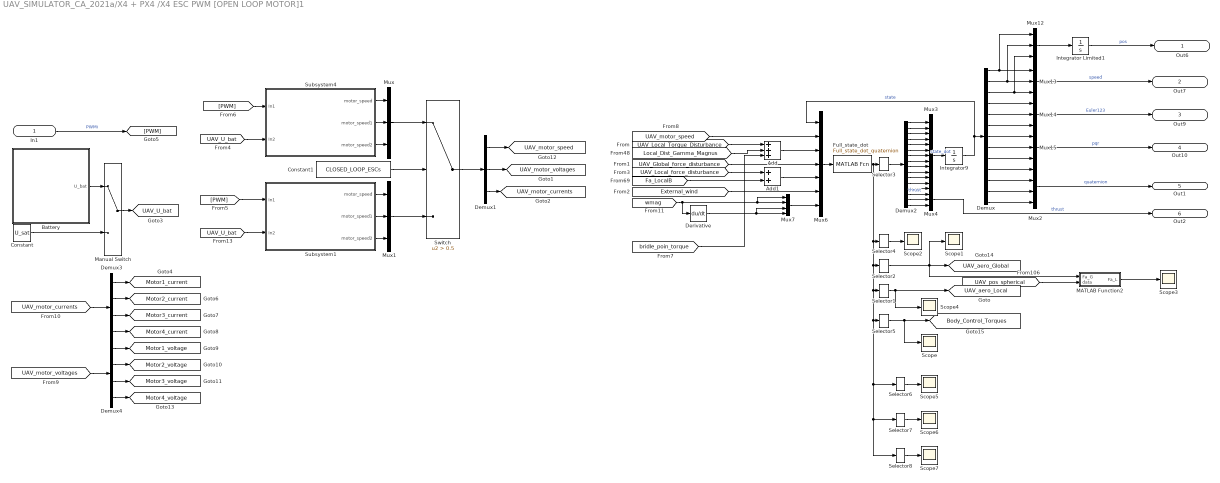
== system UAV_SIMULATOR_CA_2021a/X4 + PX4 /X4 ESC PWM [OPEN LOOP MOTOR]1 ==
  In1 : Inport
  Add : Sum  Inputs=+++
  Add1 : Sum
  Battery : Subsystem
  Constant : Constant  Value=U_sat  SampleTime=-1
  Constant1 : Constant  Value=CLOSED_LOOP_ESCs
  Demux : Demux  Outputs=13
  Demux1 : Demux  Outputs=3
  Demux2 : Demux  Outputs=16
  Demux3 : Demux
  Demux4 : Demux
  Derivative : Derivative
  Full_state_dot : MATLABFcn  MATLABFcn=Full_state_dot_quaternion  OutputDimensions=31
  Integrator Limited1 : Integrator  InitialCondition=initial_pos_conditions  LimitOutput=on  LowerSaturationLimit=[-inf -inf initial_pos_conditions(3)]
  Integrator9 : Integrator  InitialCondition=state_int
  MATLAB Function2 : MATLAB Function  TreatAsAtomicUnit=on
  Manual Switch : ManualSwitch
  Mux{,1,4,12..15} (7 alike) : Mux  Inputs=3
  Mux2 : Mux
  Mux3 : Mux  Inputs=13
  Mux6 : Mux  Inputs=7
  Mux7 : Mux
  Scope{,1..7} (8 alike) : Scope
  Selector1 : Selector  InputPortWidth=31  IndexOptions=Index vector (dialog)  Indices=[23:25]  OutputSizes=1
  Selector2 : Selector  InputPortWidth=31  IndexOptions=Index vector (dialog)  Indices=[20:22]  OutputSizes=1
  Selector3 : Selector  InputPortWidth=31  IndexOptions=Index vector (dialog)  Indices=[1:16]  OutputSizes=1
  Selector4 : Selector  InputPortWidth=31  IndexOptions=Index vector (dialog)  Indices=[17:19]  OutputSizes=1
  Selector5 : Selector  InputPortWidth=31  IndexOptions=Index vector (dialog)  Indices=[26:28]  OutputSizes=1
  Selector6 : Selector  InputPortWidth=31  IndexOptions=Index vector (dialog)  Indices=29  OutputSizes=1
  Selector7 : Selector  InputPortWidth=31  IndexOptions=Index vector (dialog)  Indices=30  OutputSizes=1
  Selector8 : Selector  InputPortWidth=31  IndexOptions=Index vector (dialog)  Indices=31  OutputSizes=1
  Subsystem1 : Subsystem
  Subsystem4 : Subsystem
  Switch : Switch  Criteria=u2 > Threshold  Threshold=0.5  SaturateOnIntegerOverflow=off  InputSameDT=off
  Out6 : Outport  VectorParamsAs1DForOutWhenUnconnected=off
  Out7 : Outport  Port=2  VectorParamsAs1DForOutWhenUnconnected=off
  Out9 : Outport  Port=3  VectorParamsAs1DForOutWhenUnconnected=off
  Out10 : Outport  Port=4  VectorParamsAs1DForOutWhenUnconnected=off
  Out1 : Outport  Port=5  VectorParamsAs1DForOutWhenUnconnected=off
  Out2 : Outport  Port=6  VectorParamsAs1DForOutWhenUnconnected=off
  tag scope: Body_Control_Torques=global, Motor1_current=global, Motor1_voltage=global, Motor2_current=global, Motor2_voltage=global, Motor3_current=global, Motor3_voltage=global, Motor4_current=global, Motor4_voltage=global, UAV_U_bat=global, UAV_aero_Global=global, UAV_aero_Local=global, UAV_motor_currents=global, UAV_motor_speed=global, UAV_motor_voltages=global
  wires:
  Mux6/1 -> Full_state_dot/1
  Demux/1 -> Mux13/1, Mux12/1
  Demux/2 -> Mux13/2, Mux12/2
  Demux/3 -> Mux12/3, Mux13/3
  Mux13/1 -> Out7/1  "speed"
  Demux/4 -> Mux14/1
  Demux/5 -> Mux14/2
  Demux/6 -> Mux14/3
  Demux/8 -> Mux15/2
  Demux/9 -> Mux15/3
  Demux/7 -> Mux15/1
  Mux14/1 -> Out9/1  "Euler123"
  Mux15/1 -> Out10/1  "pqr"
  Battery/1(U_bat) -> Manual Switch/1
  Constant/1 -> Manual Switch/2
  Demux/10 -> Mux2/1
  Demux/12 -> Mux2/3
  Demux/13 -> Mux2/4
  Demux/11 -> Mux2/2
  Mux2/1 -> Out1/1  "quaternion"
  Constant1/1 -> Switch/2
  Manual Switch/1 -> [UAV_U_bat]
  In1/1 -> [PWM]  "PWMi"
  [UAV_U_bat] -> Subsystem4/2(In2)
  [PWM] -> Subsystem1/1(In1)
  [UAV_U_bat] -> Subsystem1/2(In2)
  Subsystem4/1(motor_speed) -> Mux/1
  Subsystem4/2(motor_speed1) -> Mux/2
  Subsystem4/3(motor_speed2) -> Mux/3
  Subsystem1/2(motor_speed1) -> Mux1/2
  Subsystem1/1(motor_speed) -> Mux1/1
  Subsystem1/3(motor_speed2) -> Mux1/3
  Mux1/1 -> Switch/3
  Mux/1 -> Switch/1
  Switch/1 -> Demux1/1
  Demux1/2 -> [UAV_motor_voltages]
  Demux1/3 -> [UAV_motor_currents]
  Mux3/1 -> Integrator9/1  "state_dot"
  Demux2/13 -> Mux3/13
  Demux2/12 -> Mux3/12
  Demux2/11 -> Mux3/11
  Demux2/9 -> Mux3/9
  Demux2/8 -> Mux3/8
  Demux2/7 -> Mux3/7
  Demux2/6 -> Mux3/6
  Demux2/5 -> Mux3/5
  Demux2/4 -> Mux3/4
  Demux2/3 -> Mux3/3
  Demux2/2 -> Mux3/2
  Demux2/1 -> Mux3/1
  Demux2/14 -> Mux4/1  "thrust"
  Demux2/15 -> Mux4/2
  Demux2/16 -> Mux4/3
  Mux4/1 -> Out2/1  "thrust"
  Demux3/1 -> [Motor1_current]
  Demux3/4 -> [Motor4_current]
  Demux3/3 -> [Motor3_current]
  Demux3/2 -> [Motor2_current]
  Demux4/2 -> [Motor2_voltage]
  Demux4/3 -> [Motor3_voltage]
  Demux4/4 -> [Motor4_voltage]
  Demux4/1 -> [Motor1_voltage]
  [UAV_motor_voltages] -> Demux4/1
  [UAV_motor_currents] -> Demux3/1
  Mux12/1 -> Integrator Limited1/1
  Integrator9/1 -> Mux6/1, Demux/1  "state"
  [UAV_Local_Torque_Disturbance] -> Add/1
  Add/1 -> Mux6/3
  Mux7/1 -> Mux6/7
  [Local_Dist_Gamma_Magnus] -> Add/2
  [External_wind] -> Mux6/6
  [UAV_motor_speed] -> Mux6/2
  [UAV_Global_force_disturbance] -> Mux6/4
  Derivative/1 -> Mux7/4, Mux7/3
  [wmag] -> Derivative/1, Mux7/2, Mux7/1
  Selector3/1 -> Demux2/1
  Demux2/10 -> Mux3/10
  [UAV_Local_force_disturbance] -> Add1/1
  Add1/1 -> Mux6/5
  [Fa_LocalB] -> Add1/2
  Selector1/1 -> Scope4/1, [UAV_aero_Local]
  Selector4/1 -> Scope2/1
  Integrator Limited1/1 -> Out6/1  "pos"
  [UAV_pos_spherical] -> MATLAB Function2/2(data)
  Selector2/1 -> [UAV_aero_Global], MATLAB Function2/1(Fa_G), Scope1/1
  MATLAB Function2/1(Fa_L) -> Scope3/1
  [bridle_poin_torque] -> Add/3
  Selector5/1 -> Scope/1, [Body_Control_Torques]
  [PWM] -> Subsystem4/1(In1)
  Demux1/1 -> [UAV_motor_speed]
  Selector6/1 -> Scope5/1
  Selector7/1 -> Scope6/1
  Full_state_dot/1 -> Selector4/1, Selector2/1, Selector6/1, Selector7/1, Selector8/1, Selector5/1, Selector1/1, Selector3/1
  Selector8/1 -> Scope7/1

== system UAV_SIMULATOR_CA_2021a/Aerodynamic Forces/Magnus_Actuator/Subsystem ==
  In1 : Inport
  Gain4 : Gain  Gain=km
  Gain5 : Gain  Gain=km
  Gain6 : Gain  Gain=0.000001
  Gain7 : Gain  Gain=cQ_Magnus
  Product1 : Product
  Sum3 : Sum  Inputs=|+-
  Sum4 : Sum  Inputs=-|+|-
  Transfer Fcn2 : TransferFcn  Denominator=[L_mot R]
  Transfer Fcn3 : TransferFcn  Denominator=[Jr_Magnus 0]
  Out1 : Outport  VectorParamsAs1DForOutWhenUnconnected=off
  wires:
  Sum4/1 -> Transfer Fcn3/1
  Gain5/1 -> Sum3/2  "FEM"
  Transfer Fcn3/1 -> Product1/2, Product1/1, Out1/1, Gain6/1, Gain5/1  "W"
  Gain4/1 -> Sum4/2  "Gama_mot"
  Product1/1 -> Gain7/1
  Gain6/1 -> Sum4/3  "Gamma_fric"
  Sum3/1 -> Transfer Fcn2/1
  Gain7/1 -> Sum4/1  "Gama_load"
  Transfer Fcn2/1 -> Gain4/1  "Motor_current"
  In1/1 -> Sum3/1  "U"

== system UAV_SIMULATOR_CA_2021a/X4 + PX4 /X4 ESC PWM [OPEN LOOP MOTOR]1/Battery ==
  Add1 : Sum  Inputs=++++
  Cell {1..6} (6 alike) : Constant  Value=3.7  SampleTime=-1
  Gain : Gain  Gain=R_bat
  Mux : Mux  Inputs=6
  Selector : Selector  InputPortWidth=6  IndexOptions=Index vector (dialog)  Indices=[1:nb_battery_cells]  OutputSizes=1
  Sum : Sum  Inputs=-+|
  Sum of Elements : Sum  Inputs=+
  U_bat : Outport
  wires:
  [Motor2_current] -> Add1/2
  [Motor4_current] -> Add1/4
  Add1/1 -> Gain/1  "I_total"
  [Motor3_current] -> Add1/3
  Gain/1 -> Sum/1
  Sum/1 -> U_bat/1  "U_bat"
  Sum of Elements/1 -> Sum/2  "u_bat_max"
  [Motor1_current] -> Add1/1
  Cell 1/1 -> Mux/1
  Cell 2/1 -> Mux/2
  Cell 3/1 -> Mux/3
  Cell 4/1 -> Mux/4
  Cell 5/1 -> Mux/5
  Cell 6/1 -> Mux/6
  Mux/1 -> Selector/1
  Selector/1 -> Sum of Elements/1

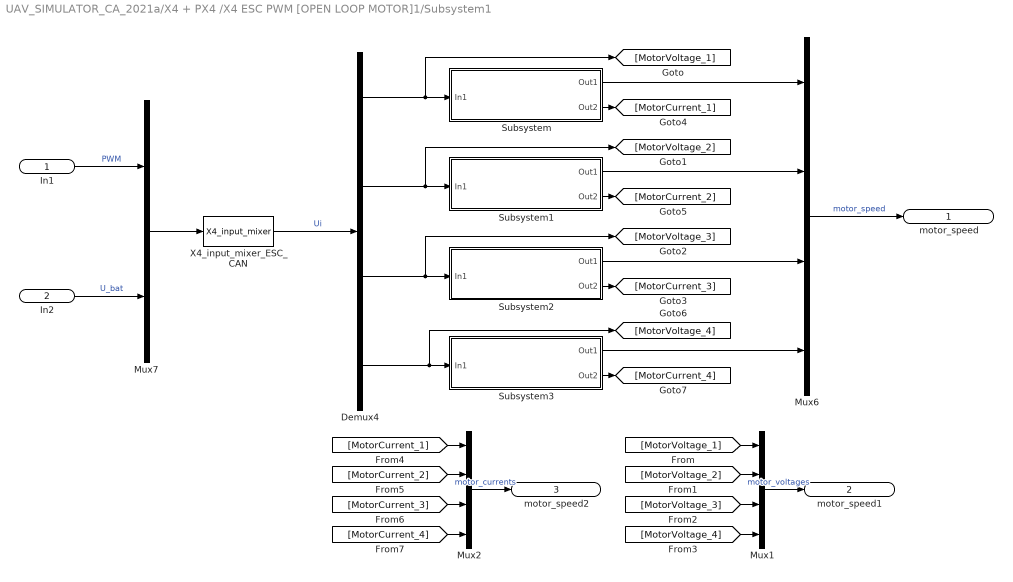
== system UAV_SIMULATOR_CA_2021a/X4 + PX4 /X4 ESC PWM [OPEN LOOP MOTOR]1/Subsystem1 ==
  In1 : Inport
  In2 : Inport  Port=2
  Demux4 : Demux
  Mux1 : Mux
  Mux2 : Mux
  Mux6 : Mux
  Mux7 : Mux  Inputs=2
  Subsystem : Subsystem
  Subsystem1 : Subsystem
  Subsystem2 : Subsystem
  Subsystem3 : Subsystem
  X4_input_mixer_ESC_CAN : MATLABFcn  MATLABFcn=X4_input_mixer  OutputDimensions=4
  motor_speed : Outport
  motor_speed1 : Outport  Port=2
  motor_speed2 : Outport  Port=3
  wires:
  Mux2/1 -> motor_speed2/1  "motor_currents"
  [MotorCurrent_4] -> Mux2/4
  [MotorCurrent_3] -> Mux2/3
  [MotorCurrent_2] -> Mux2/2
  [MotorCurrent_1] -> Mux2/1
  Demux4/4 -> [MotorVoltage_4], Subsystem3/1(In1)
  Subsystem3/1(Out1) -> Mux6/4
  Subsystem3/2(Out2) -> [MotorCurrent_4]
  Subsystem2/2(Out2) -> [MotorCurrent_3]
  Subsystem2/1(Out1) -> Mux6/3
  Demux4/3 -> [MotorVoltage_3], Subsystem2/1(In1)
  Demux4/2 -> [MotorVoltage_2], Subsystem1/1(In1)
  Subsystem1/1(Out1) -> Mux6/2
  Subsystem1/2(Out2) -> [MotorCurrent_2]
  Subsystem/2(Out2) -> [MotorCurrent_1]
  [MotorVoltage_1] -> Mux1/1
  [MotorVoltage_2] -> Mux1/2
  [MotorVoltage_3] -> Mux1/3
  [MotorVoltage_4] -> Mux1/4
  Mux1/1 -> motor_speed1/1  "motor_voltages"
  Mux6/1 -> motor_speed/1  "motor_speed"
  Subsystem/1(Out1) -> Mux6/1
  In2/1 -> Mux7/2  "U_bat"
  Demux4/1 -> [MotorVoltage_1], Subsystem/1(In1)
  In1/1 -> Mux7/1  "PWM"
  X4_input_mixer_ESC_CAN/1 -> Demux4/1  "Ui"
  Mux7/1 -> X4_input_mixer_ESC_CAN/1

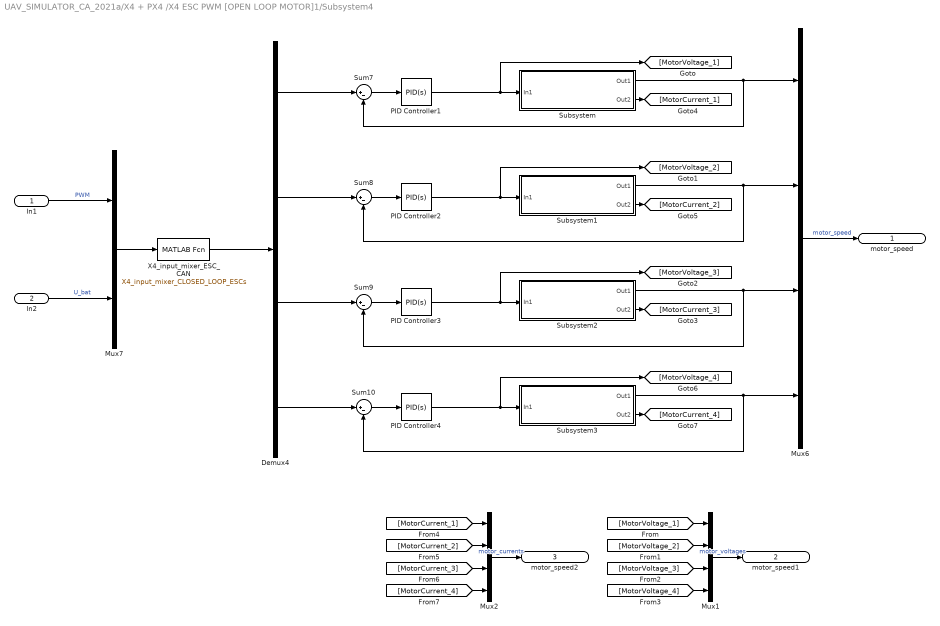
== system UAV_SIMULATOR_CA_2021a/X4 + PX4 /X4 ESC PWM [OPEN LOOP MOTOR]1/Subsystem4 ==
  In1 : Inport
  In2 : Inport  Port=2
  Demux4 : Demux
  Mux1 : Mux
  Mux2 : Mux
  Mux6 : Mux
  Mux7 : Mux  Inputs=2
  PID Controller{1..4} (4 alike) : slpidlib/PID Controller  Controller=PID  Form=Parallel  TimeDomain=Continuous-time  UseExternalTs=off  SampleTime=-1  IntegratorMethod=Forward Euler  FilterMethod=Forward Euler  ControllerParametersSource=internal  P=0.01  I=0.4  UseKiTs=off  D=0  UseExternalDerivativeSource=off  N=100  UseFilter=on  TunerSelectOption=Transfer Function Based (PID Tuner App)  InitialConditionSource=internal  InitialConditionForIntegrator=0  InitialConditionForFilter=0  DifferentiatorICPrevScaledInput=0  ExternalReset=none  TrackingMode=off  Kt=1  LimitOutput=off  SatLimitsSource=internal  UpperSaturationLimit=inf  LowerSaturationLimit=-inf  LinearizeAsGain=on  AntiWindupMode=none  Kb=1  LimitIntegrator=off  UpperIntegratorSaturationLimit=inf  LowerIntegratorSaturationLimit=-inf  POutMin=[]  POutMax=[]  IOutMin=[]  IOutMax=[]  DOutMin=[]  DOutMax=[]  NOutMin=[]  NOutMax=[]  SumOutMin=[]  SumOutMax=[]  SaturationOutMin=[]  SaturationOutMax=[]  PParamMin=[]  PParamMax=[]  IParamMin=[]  IParamMax=[]  DParamMin=[]  DParamMax=[]  NParamMin=[]  NParamMax=[]  KbParamMin=[]  KbParamMax=[]  KtParamMin=[]  KtParamMax=[]  KbOutMin=[]  KbOutMax=[]  KtOutMin=[]  KtOutMax=[]  IntegratorOutMin=[]  IntegratorOutMax=[]  FilterOutMin=[]  FilterOutMax=[]  SumI1OutMin=[]  SumI1OutMax=[]  SumI2OutMin=[]  SumI2OutMax=[]  SumI3OutMin=[]  SumI3OutMax=[]  SumI4OutMin=[]  SumI4OutMax=[]  SumDOutMin=[]  SumDOutMax=[]  DifferentiatorOutMin=[]  DifferentiatorOutMax=[]  FilterDiffOutCoefMin=[]  FilterDiffOutCoefMax=[]  ReciprocalOutMin=[]  ReciprocalOutMax=[]  SumDenOutMin=[]  SumDenOutMax=[]  SumNumOutMin=[]  SumNumOutMax=[]  DivideOutMin=[]  DivideOutMax=[]  UdiffTsProdOutMin=[]  UdiffTsProdOutMax=[]  NTsProdOutMin=[]  NTsProdOutMax=[]  UintegralTsProdOutMin=[]  UintegralTsProdOutMax=[]  UngainTsProdOutMin=[]  UngainTsProdOutMax=[]  ClampingZeroOutDataTypeStr=Inherit: Inherit via back propagation  ClampingZeroOutMin=[]  ClampingZeroOutMax=[]  FilterDenConstantOutDataTypeStr=Inherit: Inherit via back propagation  FilterDenConstantOutMin=[]  FilterDenConstantOutMax=[]  PCopyOutDataTypeStr=Inherit: Inherit via back propagation  PCopyOutMin=[]  PCopyOutMax=[]  NCopyOutDataTypeStr=Inherit: Inherit via back propagation  NCopyOutMin=[]  NCopyOutMax=[]  IntegratorContinuousStateAttributes=''  IntegratorStateMustResolveToSignalObject=off  IntegratorRTWStateStorageClass=Auto  FilterContinuousStateAttributes=''  FilterStateMustResolveToSignalObject=off  FilterRTWStateStorageClass=Auto  ParallelPVariant=InternalParameters  IdealPVariant=Disabled  IVariant=InternalParameters  DVariant=InternalParameters  IntegratorVariant=Continuous  SatVariant=Disabled  AWVariant=Passthrough  PCopyVariant=Disabled  TRVariant=Disabled  FdbkBlocksVariant=Forward  IdealPFdbkVariant=Disabled  SatFdbkVariant=Disabled  DerivativeFilterVariant=ContFilter  NVariant=InternalParameters  NCopyVariant=Disabled  FilterICVariant=InternalICsFilter  IntegratorICVariant=InternalICs  ExternalResetVariant=Disabled  TRSumVariant=Passthrough  SumFdbkVariant=Disabled  SumVariant=Sum_PID  TsampFilterVariant=InternalTs  TsampNgainVariant=Passthrough  TsampIntegralVariant=Disabled_SignalSpec  ExternalSaturationOutDataTypeStr=Inherit: Same as second input  DerivativeSourceVariant=ErrorSignal
  Subsystem : Subsystem
  Subsystem1 : Subsystem
  Subsystem2 : Subsystem
  Subsystem3 : Subsystem
  Sum{7..10} (4 alike) : Sum  Inputs=|+-
  X4_input_mixer_ESC_CAN : MATLABFcn  MATLABFcn=X4_input_mixer_CLOSED_LOOP_ESCs  OutputDimensions=4
  motor_speed : Outport
  motor_speed1 : Outport  Port=2
  motor_speed2 : Outport  Port=3
  wires:
  Demux4/2 -> Sum8/1
  Demux4/4 -> Sum10/1
  Sum8/1 -> PID Controller2/1
  Mux7/1 -> X4_input_mixer_ESC_CAN/1
  Sum7/1 -> PID Controller1/1
  X4_input_mixer_ESC_CAN/1 -> Demux4/1
  Sum9/1 -> PID Controller3/1
  In1/1 -> Mux7/1  "PWM"
  Demux4/1 -> Sum7/1
  PID Controller1/1 -> [MotorVoltage_1], Subsystem/1(In1)
  In2/1 -> Mux7/2  "U_bat"
  Subsystem/1(Out1) -> Sum7/2, Mux6/1
  Mux6/1 -> motor_speed/1  "motor_speed"
  Demux4/3 -> Sum9/1
  Mux1/1 -> motor_speed1/1  "motor_voltages"
  [MotorVoltage_4] -> Mux1/4
  [MotorVoltage_3] -> Mux1/3
  [MotorVoltage_2] -> Mux1/2
  [MotorVoltage_1] -> Mux1/1
  Subsystem/2(Out2) -> [MotorCurrent_1]
  Subsystem1/2(Out2) -> [MotorCurrent_2]
  Subsystem1/1(Out1) -> Sum8/2, Mux6/2
  PID Controller2/1 -> Subsystem1/1(In1), [MotorVoltage_2]
  PID Controller3/1 -> [MotorVoltage_3], Subsystem2/1(In1)
  Subsystem2/1(Out1) -> Sum9/2, Mux6/3
  Subsystem2/2(Out2) -> [MotorCurrent_3]
  Subsystem3/2(Out2) -> [MotorCurrent_4]
  Subsystem3/1(Out1) -> Sum10/2, Mux6/4
  PID Controller4/1 -> Subsystem3/1(In1), [MotorVoltage_4]
  Sum10/1 -> PID Controller4/1
  [MotorCurrent_1] -> Mux2/1
  [MotorCurrent_2] -> Mux2/2
  [MotorCurrent_3] -> Mux2/3
  [MotorCurrent_4] -> Mux2/4
  Mux2/1 -> motor_speed2/1  "motor_currents"

== system UAV_SIMULATOR_CA_2021a/X4 + PX4 /X4 ESC PWM [OPEN LOOP MOTOR]1/Subsystem1/Subsystem ==
  In1 : Inport
  Gain4 : Gain  Gain=km
  Gain5 : Gain  Gain=km
  Gain6 : Gain  Gain=0.000001
  Gain7 : Gain  Gain=cQ
  Product1 : Product
  Sum3 : Sum  Inputs=|+-
  Sum4 : Sum  Inputs=-|+|-
  Transfer Fcn2 : TransferFcn  Denominator=[L_mot R]
  Transfer Fcn3 : TransferFcn  Denominator=[Jr 0]
  Out1 : Outport  VectorParamsAs1DForOutWhenUnconnected=off
  Out2 : Outport  Port=2  VectorParamsAs1DForOutWhenUnconnected=off
  wires:
  In1/1 -> Sum3/1  "U"
  Transfer Fcn2/1 -> Gain4/1, Out2/1  "Motor_current"
  Gain7/1 -> Sum4/1  "Gama_load"
  Sum3/1 -> Transfer Fcn2/1
  Gain6/1 -> Sum4/3  "Gamma_fric"
  Product1/1 -> Gain7/1
  Gain4/1 -> Sum4/2  "Gama_mot"
  Transfer Fcn3/1 -> Gain5/1, Gain6/1, Out1/1, Product1/1, Product1/2  "W"
  Gain5/1 -> Sum3/2  "FEM"
  Sum4/1 -> Transfer Fcn3/1

== system UAV_SIMULATOR_CA_2021a/X4 + PX4 /X4 ESC PWM [OPEN LOOP MOTOR]1/Subsystem1/Subsystem1 ==
  In1 : Inport
  Gain4 : Gain  Gain=km
  Gain5 : Gain  Gain=km
  Gain6 : Gain  Gain=0.000001
  Gain7 : Gain  Gain=cQ
  Product1 : Product
  Sum3 : Sum  Inputs=|+-
  Sum4 : Sum  Inputs=-|+|-
  Transfer Fcn2 : TransferFcn  Denominator=[L_mot R]
  Transfer Fcn3 : TransferFcn  Denominator=[Jr 0]
  Out1 : Outport  VectorParamsAs1DForOutWhenUnconnected=off
  Out2 : Outport  Port=2  VectorParamsAs1DForOutWhenUnconnected=off
  wires:
  Sum4/1 -> Transfer Fcn3/1
  Gain5/1 -> Sum3/2  "FEM"
  Transfer Fcn3/1 -> Product1/2, Product1/1, Out1/1, Gain6/1, Gain5/1  "W"
  Gain4/1 -> Sum4/2  "Gama_mot"
  Product1/1 -> Gain7/1
  Gain6/1 -> Sum4/3  "Gamma_fric"
  Sum3/1 -> Transfer Fcn2/1
  Gain7/1 -> Sum4/1  "Gama_load"
  Transfer Fcn2/1 -> Out2/1, Gain4/1  "Motor_current"
  In1/1 -> Sum3/1  "U"

== system UAV_SIMULATOR_CA_2021a/X4 + PX4 /X4 ESC PWM [OPEN LOOP MOTOR]1/Subsystem1/Subsystem2 ==
  In1 : Inport
  Gain4 : Gain  Gain=km
  Gain5 : Gain  Gain=km
  Gain6 : Gain  Gain=0.000001
  Gain7 : Gain  Gain=cQ
  Product1 : Product
  Sum3 : Sum  Inputs=|+-
  Sum4 : Sum  Inputs=-|+|-
  Transfer Fcn2 : TransferFcn  Denominator=[L_mot R]
  Transfer Fcn3 : TransferFcn  Denominator=[Jr 0]
  Out1 : Outport  VectorParamsAs1DForOutWhenUnconnected=off
  Out2 : Outport  Port=2  VectorParamsAs1DForOutWhenUnconnected=off
  wires:
  In1/1 -> Sum3/1  "U"
  Transfer Fcn2/1 -> Gain4/1, Out2/1  "Motor_current"
  Gain7/1 -> Sum4/1  "Gama_load"
  Sum3/1 -> Transfer Fcn2/1
  Gain6/1 -> Sum4/3  "Gamma_fric"
  Product1/1 -> Gain7/1
  Gain4/1 -> Sum4/2  "Gama_mot"
  Transfer Fcn3/1 -> Gain5/1, Gain6/1, Out1/1, Product1/1, Product1/2  "W"
  Gain5/1 -> Sum3/2  "FEM"
  Sum4/1 -> Transfer Fcn3/1

== system UAV_SIMULATOR_CA_2021a/X4 + PX4 /X4 ESC PWM [OPEN LOOP MOTOR]1/Subsystem1/Subsystem3 ==
  In1 : Inport
  Gain4 : Gain  Gain=km
  Gain5 : Gain  Gain=km
  Gain6 : Gain  Gain=0.000001
  Gain7 : Gain  Gain=cQ
  Product1 : Product
  Sum3 : Sum  Inputs=|+-
  Sum4 : Sum  Inputs=-|+|-
  Transfer Fcn2 : TransferFcn  Denominator=[L_mot R]
  Transfer Fcn3 : TransferFcn  Denominator=[Jr 0]
  Out1 : Outport  VectorParamsAs1DForOutWhenUnconnected=off
  Out2 : Outport  Port=2  VectorParamsAs1DForOutWhenUnconnected=off
  wires:
  Sum4/1 -> Transfer Fcn3/1
  Gain5/1 -> Sum3/2  "FEM"
  Transfer Fcn3/1 -> Product1/2, Product1/1, Out1/1, Gain6/1, Gain5/1  "W"
  Gain4/1 -> Sum4/2  "Gama_mot"
  Product1/1 -> Gain7/1
  Gain6/1 -> Sum4/3  "Gamma_fric"
  Sum3/1 -> Transfer Fcn2/1
  Gain7/1 -> Sum4/1  "Gama_load"
  Transfer Fcn2/1 -> Out2/1, Gain4/1  "Motor_current"
  In1/1 -> Sum3/1  "U"

== system UAV_SIMULATOR_CA_2021a/X4 + PX4 /X4 ESC PWM [OPEN LOOP MOTOR]1/Subsystem4/Subsystem ==
  In1 : Inport
  Gain4 : Gain  Gain=km
  Gain5 : Gain  Gain=km
  Gain6 : Gain  Gain=0.000001
  Gain7 : Gain  Gain=cQ
  Product1 : Product
  Sum3 : Sum  Inputs=|+-
  Sum4 : Sum  Inputs=-|+|-
  Transfer Fcn2 : TransferFcn  Denominator=[L_mot R]
  Transfer Fcn3 : TransferFcn  Denominator=[Jr 0]
  Out1 : Outport  VectorParamsAs1DForOutWhenUnconnected=off
  Out2 : Outport  Port=2  VectorParamsAs1DForOutWhenUnconnected=off
  wires:
  Sum4/1 -> Transfer Fcn3/1
  Gain5/1 -> Sum3/2  "FEM"
  Transfer Fcn3/1 -> Product1/2, Product1/1, Out1/1, Gain6/1, Gain5/1  "W"
  Gain4/1 -> Sum4/2  "Gama_mot"
  Product1/1 -> Gain7/1
  Gain6/1 -> Sum4/3  "Gamma_fric"
  Sum3/1 -> Transfer Fcn2/1
  Gain7/1 -> Sum4/1  "Gama_load"
  Transfer Fcn2/1 -> Out2/1, Gain4/1  "Motor_current"
  In1/1 -> Sum3/1  "U"

== system UAV_SIMULATOR_CA_2021a/X4 + PX4 /X4 ESC PWM [OPEN LOOP MOTOR]1/Subsystem4/Subsystem1 ==
  In1 : Inport
  Gain4 : Gain  Gain=km
  Gain5 : Gain  Gain=km
  Gain6 : Gain  Gain=0.000001
  Gain7 : Gain  Gain=cQ
  Product1 : Product
  Sum3 : Sum  Inputs=|+-
  Sum4 : Sum  Inputs=-|+|-
  Transfer Fcn2 : TransferFcn  Denominator=[L_mot R]
  Transfer Fcn3 : TransferFcn  Denominator=[Jr 0]
  Out1 : Outport  VectorParamsAs1DForOutWhenUnconnected=off
  Out2 : Outport  Port=2  VectorParamsAs1DForOutWhenUnconnected=off
  wires:
  In1/1 -> Sum3/1  "U"
  Transfer Fcn2/1 -> Gain4/1, Out2/1  "Motor_current"
  Gain7/1 -> Sum4/1  "Gama_load"
  Sum3/1 -> Transfer Fcn2/1
  Gain6/1 -> Sum4/3  "Gamma_fric"
  Product1/1 -> Gain7/1
  Gain4/1 -> Sum4/2  "Gama_mot"
  Transfer Fcn3/1 -> Gain5/1, Gain6/1, Out1/1, Product1/1, Product1/2  "W"
  Gain5/1 -> Sum3/2  "FEM"
  Sum4/1 -> Transfer Fcn3/1
